simulink model "current_loop_cc"  (R2026b)
settings: Solver=VariableStepAuto  StopTime=3e-3  MaxStep=1e-6
values from neighbouring files (symbols this model uses):
  L = 0.88e-3    (= 0.00088)    [current_loop_design.m]
  R = 3.21    [current_loop_design.m]
  Ts = 50e-6    (= 5e-05)    [current_loop_design.m]
undefined symbols (not defined in the file or in its folder): SampleTime
settings Model: Creator=22101  LastModifiedBy=22101
settings SFSimCC: SimCustomHeaderCode="#include \"pi_sim.h\""  SimCustomInitializer=pi_sim_reset();
settings SFSimCC: SimUserIncludeDirs=|
  | cc
  | ../core
settings SFSimCC: SimUserSources=|
  | cc/pi_sim.c
  | ../core/pi.c

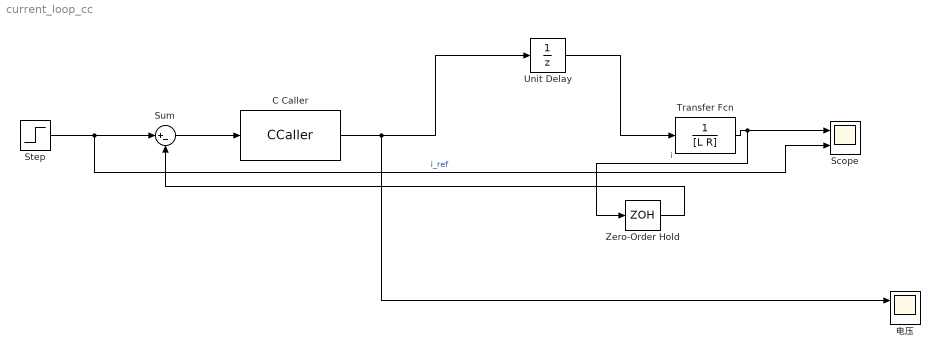
== system current_loop_cc ==
  C Caller : CCaller  FunctionName=pi_sim_step  PortSpecificationStruct="%)30     .    8 H   8    (     @         %    \"     8    !     0         %  0 \"0    $    _    07)G3F%M90  4&]R=$YA;64 4V-O<&4     26YD97@     5'EP90      4VEZ90      27-';&]B86P   X    P    !@    @    $          4    (     0    ,    !         !   P!O=70 #@   #     &    \"     0         !0    @    !     P    $         $  # &]U=  .    .     8    (    !          %    \"     $    &     0         0   ...(+3204 chars)"  SampleTime=SampleTime  kp=Kp  ki=Ki  ts=Ts  out_max=Vmax  SampleTime=Ts
  Scope : Scope  NumInputPorts=2
      settings: ActiveDisplayYMinimum=-0.47179168936075355  ActiveDisplayYMaximum=2.3027732984901839
  Step : Step  Time=0  FinalValue=2  SampleTime=0
  Sum : Sum  Inputs=|+-
  Transfer Fcn : TransferFcn  Denominator=[L R]
  Unit Delay : UnitDelay  SampleTime=Ts
  Zero-Order Hold : ZeroOrderHold  SampleTime=Ts
  电压 : Scope  NumInputPorts=2
      settings: ActiveDisplayYMinimum=-0.866025388240814  ActiveDisplayYMaximum=7.7942284941673279
  wires:
  Step/1 -> Scope/2, Sum/1  "i_ref"
  Transfer Fcn/1 -> Zero-Order Hold/1, Scope/1  "i"
  Unit Delay/1 -> Transfer Fcn/1
  Zero-Order Hold/1 -> Sum/2
  Sum/1 -> C Caller/1
  C Caller/1 -> 电压/1, Unit Delay/1
